simulink model "Exp02"  (R2024b)
settings: Solver=VariableStepAuto  StartTime=0.0  StopTime=0.02  RelTol=1e-3
libraries: spsACVoltageSourceLib x3, spsGroundLib x3, spsRMSLib x3, eePowerMeasurement x2, spsVoltageMeasurementLib x2, spsCurrentMeasurementLib x1, spsThreePhaseSeriesRLCBranchLib x1, spsThreePhaseVIMeasurementLib x1, sps_lib x1
settings Model: Creator=HP  LastModifiedBy=HP

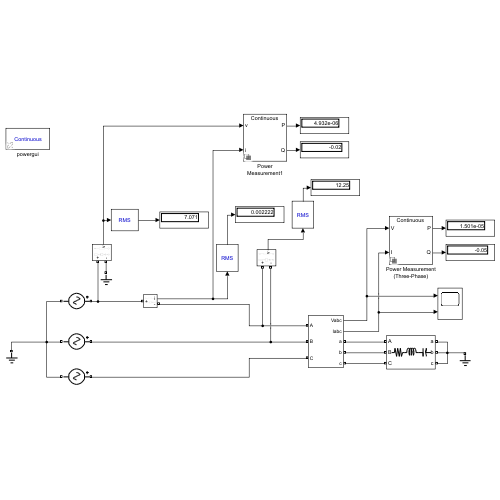
[thumbnail: Simulink's stored preview of the top-level diagram]
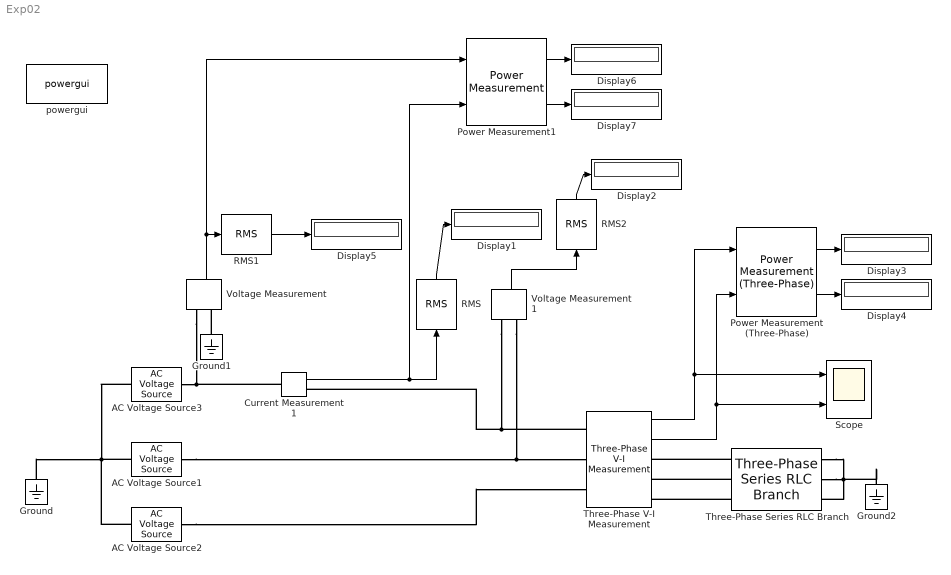
== system Exp02 ==
  AC Voltage Source1 : spsACVoltageSourceLib/AC Voltage Source  Amplitude=10  Phase=-120  Frequency=50  SampleTime=0  Measurements=None  BusType=swing  Pref=10e3  Qref=0  Qmin=-inf  Qmax=+inf
  AC Voltage Source2 : spsACVoltageSourceLib/AC Voltage Source  Amplitude=10  Phase=120  Frequency=50  SampleTime=0  Measurements=None  BusType=swing  Pref=10e3  Qref=0  Qmin=-inf  Qmax=+inf
  AC Voltage Source3 : spsACVoltageSourceLib/AC Voltage Source  Amplitude=10  Phase=0  Frequency=50  SampleTime=0  Measurements=None  BusType=swing  Pref=10e3  Qref=0  Qmin=-inf  Qmax=+inf
  Current Measurement1 : spsCurrentMeasurementLib/Current Measurement  PhasorSimulation=off  OutputType=Complex  PSBequivalent=0
  Display{1..7} (7 alike) : Display
      Display4 settings: Format=bank
      Display7 settings: Format=bank
  Ground : spsGroundLib/Ground  LConnTagsString=a
  Ground1 : spsGroundLib/Ground  LConnTagsString=a
  Ground2 : spsGroundLib/Ground  LConnTagsString=a
  Power Measurement1 : eePowerMeasurement/Power Measurement  LabelModeActiveChoice=Continuous  F=50  K=[1]  Ts=0
  Power Measurement (Three-Phase) : eePowerMeasurement/Power Measurement (Three-Phase)  LabelModeActiveChoice=Continuous  F=50  K=[1]  Seq=Positive  Ts=0
  RMS : spsRMSLib/RMS  TrueRMS=on  Freq=50  RMSInit=120  Ts=0
  RMS1 : spsRMSLib/RMS  TrueRMS=on  Freq=50  RMSInit=120  Ts=0
  RMS2 : spsRMSLib/RMS  TrueRMS=on  Freq=50  RMSInit=120  Ts=0
  Scope : Scope  NumInputPorts=2
  Three-Phase Series RLC Branch : spsThreePhaseSeriesRLCBranchLib/Three-Phase Series RLC Branch  LConnTagsString=A|B|C  RConnTagsString=A|B|C  BranchType=RLC  Resistance=1  Inductance=1e-3  Capacitance=1e-6  Measurements=None
  Three-Phase V-I Measurement : spsThreePhaseVIMeasurementLib/Three-Phase V-I Measurement  VoltageMeasurement=phase-to-ground  SetLabelV=off  LabelV=Vabc  Vpu=off  VpuLL=off  CurrentMeasurement=yes  SetLabelI=off  LabelI=Iabc  Ipu=off  Pbase=100e6  Vbase=500e3  OutputType=Complex  PhasorSimulation=off  PSBequivalent=0
  Voltage Measurement : spsVoltageMeasurementLib/Voltage Measurement  PhasorSimulation=off  OutputType=Complex  PSBequivalent=0
  Voltage Measurement1 : spsVoltageMeasurementLib/Voltage Measurement  PhasorSimulation=off  OutputType=Complex  PSBequivalent=0
  powergui : sps_lib/powergui  Priority=1  SimulationMode=Continuous  SampleTime=50e-6  frequency=60  Iterations=50  frequencyindice=50  Pbase=100e6  ErrMax=1e-4  UnitsV=kV  UnitsW=MW  buscounter=0  FunctionMessages=off  echomessages=off  EnableUseOfTLC=off  CurrentSourceSwitches=off  DisableSnubberDevices=off  DisableRonSwitches=off  DisableVfSwitches=off  DisplayEquations=off  AutomaticDiscreteSolvers=off  SolverType=Tustin/Backward Euler (TBE)  Interpol=off  ExternalGateDelay=off  methode=off  Ts=100  x0status=blocks  SPID=on  SwTol=0  HookPort=off  NonlinearTolerance=1e-4  nMaxIteration=100  ContinueOnMaxIteration=off  RestoreLinks=warning  ResistiveCurrentMeasurement=off  Frange=[0:2:500]  Ylog=off  Xlog=on  ShowGrid=off  save=off  variable=ZData  structure=0  ZoomFFT=off  StartTime=0.0  cycles=1  DisplayStyle=1  fundamental=60  FreqAxis=off  MaxFrequency=1000  frequencyindicesteady=1  RmsSteady=1  display=off
  wires:
  RMS/1 -> Display1/1
  Three-Phase V-I Measurement/1 -> Power Measurement (Three-Phase)/1, Scope/1
  Three-Phase V-I Measurement/2 -> Power Measurement (Three-Phase)/2, Scope/2
  Power Measurement (Three-Phase)/2 -> Display4/1
  Power Measurement (Three-Phase)/1 -> Display3/1
  Current Measurement1/1 -> Power Measurement1/2, RMS/1
  Power Measurement1/1 -> Display6/1
  Power Measurement1/2 -> Display7/1
  Voltage Measurement1/1 -> RMS2/1
  RMS2/1 -> Display2/1
  RMS1/1 -> Display5/1
  Voltage Measurement/1 -> Power Measurement1/1, RMS1/1
  connections:
  Ground/LConn1 -- AC Voltage Source1/LConn1 -- AC Voltage Source2/LConn1 -- AC Voltage Source3/LConn1
  Current Measurement1/LConn1 -- AC Voltage Source3/RConn1 -- Voltage Measurement/LConn1
  Three-Phase V-I Measurement/LConn1 -- Voltage Measurement1/LConn1 -- Current Measurement1/RConn1
  AC Voltage Source1/RConn1 -- Three-Phase V-I Measurement/LConn2 -- Voltage Measurement1/LConn2
  AC Voltage Source2/RConn1 -- Three-Phase V-I Measurement/LConn3
  Three-Phase Series RLC Branch/LConn1 -- Three-Phase V-I Measurement/RConn1
  Three-Phase Series RLC Branch/LConn2 -- Three-Phase V-I Measurement/RConn2
  Three-Phase Series RLC Branch/LConn3 -- Three-Phase V-I Measurement/RConn3
  Ground1/LConn1 -- Voltage Measurement/LConn2
  Three-Phase Series RLC Branch/RConn1 -- Three-Phase Series RLC Branch/RConn3 -- Ground2/LConn1 -- Three-Phase Series RLC Branch/RConn2
